simulink model "mijo"  (R2026b)
settings: Solver=VariableStepAuto  StopTime=15.0  MaxStep=1E-2
libraries: slpidlib x2
settings Model: LastModifiedBy=Emiliano
settings DataIOCC: DSMLogging=off  ReturnWorkspaceOutputs=off  SaveOutput=off  SignalLogging=off  TimeSaveName=t
settings DebuggingCC: AlgebraicLoopMsg=none  ArtificialAlgebraicLoopMsg=none  MaxConsecutiveZCsMsg=none

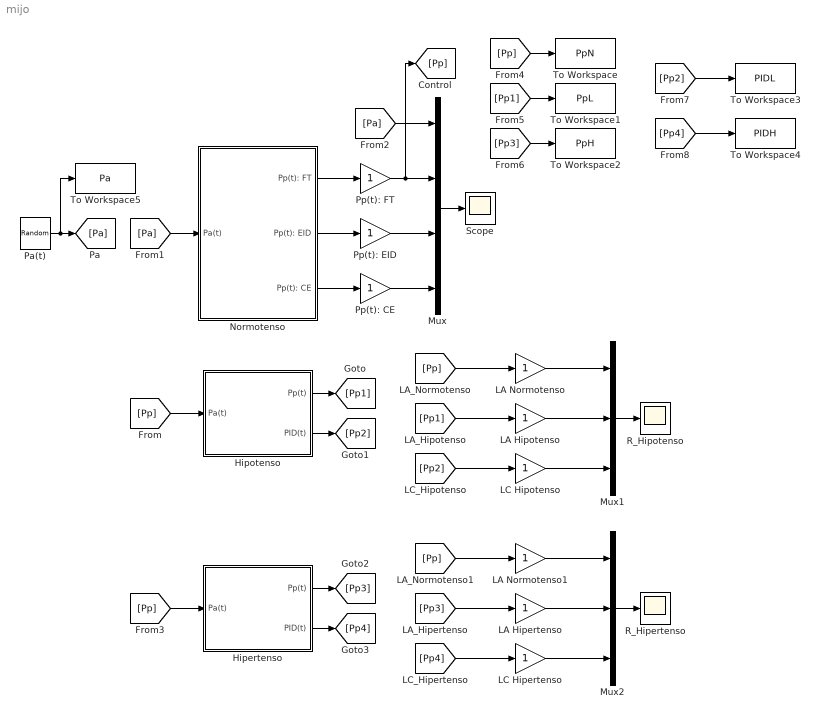
== system mijo ==
  Hipertenso : Subsystem
  Hipotenso : Subsystem
  LA Hipertenso : Gain
  LA Hipotenso : Gain
  LA Normotenso : Gain
  LA Normotenso1 : Gain
  LC Hipertenso : Gain
  LC Hipotenso : Gain
  Mux : Mux
  Mux1 : Mux  Inputs=3
  Mux2 : Mux  Inputs=3
  Normotenso : Subsystem
  Pa(t) : UniformRandomNumber  Minimum=-0.2  Seed=106  SampleTime=0.1
  Pp(t): CE : Gain
  Pp(t): EID : Gain
  Pp(t): FT : Gain
  R_Hipertenso : Scope
      settings: ActiveDisplayYMinimum=-0.45088607175795514  ActiveDisplayYMaximum=1.1087942936567985  DataLoggingVariableName=ScopeData2
  R_Hipotenso : Scope
      settings: ActiveDisplayYMinimum=0.091688488718673522  ActiveDisplayYMaximum=1.8821623827103118
  Scope : Scope
      settings: ActiveDisplayYMinimum=-0.51846261387700343  ActiveDisplayYMaximum=1.1468505763363619
  To Workspace : ToWorkspace  VariableName=PpN  SampleTime=-1
  To Workspace1 : ToWorkspace  VariableName=PpL  SampleTime=-1
  To Workspace2 : ToWorkspace  VariableName=PpH  SampleTime=-1
  To Workspace3 : ToWorkspace  VariableName=PIDL  SampleTime=-1
  To Workspace4 : ToWorkspace  VariableName=PIDH  SampleTime=-1
  To Workspace5 : ToWorkspace  VariableName=Pa  SampleTime=-1
  wires:
  Mux/1 -> Scope/1
  Normotenso/2(Pp(t): EID) -> Pp(t): EID/1
  Normotenso/3(Pp(t): CE) -> Pp(t): CE/1
  Normotenso/1(Pp(t): FT) -> Pp(t): FT/1
  Pp(t): FT/1 -> [Pp], Mux/2
  Pp(t): EID/1 -> Mux/3
  Pp(t): CE/1 -> Mux/4
  Pa(t)/1 -> To Workspace5/1, [Pa]
  [Pa] -> Normotenso/1(Pa(t))
  [Pa] -> Mux/1
  [Pp] -> Hipotenso/1(Pa(t))
  Hipotenso/1(Pp(t)) -> [Pp1]
  Hipotenso/2(PID(t)) -> [Pp2]
  [Pp] -> LA Normotenso/1
  [Pp1] -> LA Hipotenso/1
  [Pp2] -> LC Hipotenso/1
  Mux1/1 -> R_Hipotenso/1
  LA Normotenso/1 -> Mux1/1
  LA Hipotenso/1 -> Mux1/2
  LC Hipotenso/1 -> Mux1/3
  Hipertenso/2(PID(t)) -> [Pp4]
  Hipertenso/1(Pp(t)) -> [Pp3]
  [Pp] -> Hipertenso/1(Pa(t))
  LA Hipertenso/1 -> Mux2/2
  LA Normotenso1/1 -> Mux2/1
  Mux2/1 -> R_Hipertenso/1
  LC Hipertenso/1 -> Mux2/3
  [Pp4] -> LC Hipertenso/1
  [Pp3] -> LA Hipertenso/1
  [Pp] -> LA Normotenso1/1
  [Pp] -> To Workspace/1
  [Pp1] -> To Workspace1/1
  [Pp3] -> To Workspace2/1
  [Pp2] -> To Workspace3/1
  [Pp4] -> To Workspace4/1

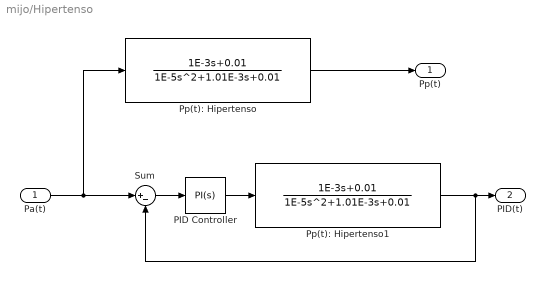
== system mijo/Hipertenso ==
  Pa(t) : Inport
  PID Controller : slpidlib/PID Controller  Controller=PI  Form=Parallel  TimeDomain=Continuous-time  UseExternalTs=off  SampleTime=-1  IntegratorMethod=Forward Euler  FilterMethod=Forward Euler  ControllerParametersSource=internal  P=205.8701  I=74187.5742  UseKiTs=off  D=0  UseExternalDerivativeSource=off  N=100  UseFilter=on  TunerSelectOption=Transfer Function Based (PID Tuner App)  InitialConditionSource=internal  InitialConditionForIntegrator=0  InitialConditionForFilter=0  DifferentiatorICPrevScaledInput=0  ExternalReset=none  TrackingMode=off  Kt=1  LimitOutput=off  SatLimitsSource=internal  UpperSaturationLimit=inf  LowerSaturationLimit=-inf  LinearizeAsGain=on  AntiWindupMode=none  Kb=1  LimitIntegrator=off  UpperIntegratorSaturationLimit=inf  LowerIntegratorSaturationLimit=-inf  POutMin=[]  POutMax=[]  IOutMin=[]  IOutMax=[]  DOutMin=[]  DOutMax=[]  NOutMin=[]  NOutMax=[]  SumOutMin=[]  SumOutMax=[]  SaturationOutMin=[]  SaturationOutMax=[]  PParamMin=[]  PParamMax=[]  IParamMin=[]  IParamMax=[]  DParamMin=[]  DParamMax=[]  NParamMin=[]  NParamMax=[]  KbParamMin=[]  KbParamMax=[]  KtParamMin=[]  KtParamMax=[]  KbOutMin=[]  KbOutMax=[]  KtOutMin=[]  KtOutMax=[]  IntegratorOutMin=[]  IntegratorOutMax=[]  FilterOutMin=[]  FilterOutMax=[]  SumI1OutMin=[]  SumI1OutMax=[]  SumI2OutMin=[]  SumI2OutMax=[]  SumI3OutMin=[]  SumI3OutMax=[]  SumI4OutMin=[]  SumI4OutMax=[]  SumDOutMin=[]  SumDOutMax=[]  DifferentiatorOutMin=[]  DifferentiatorOutMax=[]  FilterDiffOutCoefMin=[]  FilterDiffOutCoefMax=[]  ReciprocalOutMin=[]  ReciprocalOutMax=[]  SumDenOutMin=[]  SumDenOutMax=[]  SumNumOutMin=[]  SumNumOutMax=[]  DivideOutMin=[]  DivideOutMax=[]  UdiffTsProdOutMin=[]  UdiffTsProdOutMax=[]  NTsProdOutMin=[]  NTsProdOutMax=[]  UintegralTsProdOutMin=[]  UintegralTsProdOutMax=[]  UngainTsProdOutMin=[]  UngainTsProdOutMax=[]  ClampingZeroOutDataTypeStr=Inherit: Inherit via back propagation  ClampingZeroOutMin=[]  ClampingZeroOutMax=[]  FilterDenConstantOutDataTypeStr=Inherit: Inherit via back propagation  FilterDenConstantOutMin=[]  FilterDenConstantOutMax=[]  PCopyOutDataTypeStr=Inherit: Inherit via back propagation  PCopyOutMin=[]  PCopyOutMax=[]  NCopyOutDataTypeStr=Inherit: Inherit via back propagation  NCopyOutMin=[]  NCopyOutMax=[]  IntegratorContinuousStateAttributes=''  IntegratorStateMustResolveToSignalObject=off  IntegratorRTWStateStorageClass=Auto  FilterContinuousStateAttributes=''  FilterStateMustResolveToSignalObject=off  FilterRTWStateStorageClass=Auto  ParallelPVariant=InternalParameters  IdealPVariant=Disabled  IVariant=InternalParameters  DVariant=Disabled  IntegratorVariant=Continuous  SatVariant=Disabled  AWVariant=Passthrough  PCopyVariant=Disabled  TRVariant=Disabled  FdbkBlocksVariant=Forward  IdealPFdbkVariant=Disabled  SatFdbkVariant=Disabled  DerivativeFilterVariant=Disabled  NVariant=Disabled  NCopyVariant=Disabled_SignalSpec  FilterICVariant=Disabled  IntegratorICVariant=InternalICs  ExternalResetVariant=Disabled  TRSumVariant=Passthrough  SumFdbkVariant=Disabled  SumVariant=Sum_PI  TsampFilterVariant=InternalTs  TsampNgainVariant=Passthrough  TsampIntegralVariant=Disabled_SignalSpec  ExternalSaturationOutDataTypeStr=Inherit: Same as second input  DerivativeSourceVariant=Disabled  PreIntVariant=InternalPreInt
  Pp(t): Hipertenso : TransferFcn  Numerator=[1E-3,0.01]  Denominator=[1E-5,1.01E-3,0.01]
  Pp(t): Hipertenso1 : TransferFcn  Numerator=[1E-3,0.01]  Denominator=[1E-5,1.01E-3,0.01]
  Sum : Sum  Inputs=|+-
  Pp(t) : Outport
  PID(t) : Outport  Port=2
  wires:
  Pa(t)/1 -> Pp(t): Hipertenso/1, Sum/1
  PID Controller/1 -> Pp(t): Hipertenso1/1
  Sum/1 -> PID Controller/1
  Pp(t): Hipertenso1/1 -> Sum/2, PID(t)/1
  Pp(t): Hipertenso/1 -> Pp(t)/1

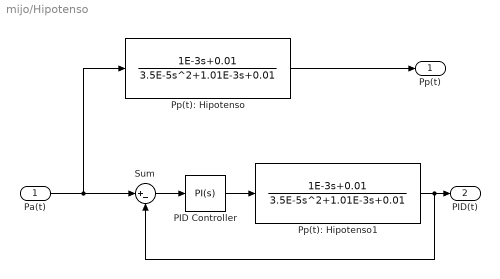
== system mijo/Hipotenso ==
  Pa(t) : Inport
  PID Controller : slpidlib/PID Controller  Controller=PI  Form=Parallel  TimeDomain=Continuous-time  UseExternalTs=off  SampleTime=-1  IntegratorMethod=Forward Euler  FilterMethod=Forward Euler  ControllerParametersSource=internal  P=174.4048  I=15212.346  UseKiTs=off  D=0  UseExternalDerivativeSource=off  N=100  UseFilter=on  TunerSelectOption=Transfer Function Based (PID Tuner App)  InitialConditionSource=internal  InitialConditionForIntegrator=0  InitialConditionForFilter=0  DifferentiatorICPrevScaledInput=0  ExternalReset=none  TrackingMode=off  Kt=1  LimitOutput=off  SatLimitsSource=internal  UpperSaturationLimit=inf  LowerSaturationLimit=-inf  LinearizeAsGain=on  AntiWindupMode=none  Kb=1  LimitIntegrator=off  UpperIntegratorSaturationLimit=inf  LowerIntegratorSaturationLimit=-inf  POutMin=[]  POutMax=[]  IOutMin=[]  IOutMax=[]  DOutMin=[]  DOutMax=[]  NOutMin=[]  NOutMax=[]  SumOutMin=[]  SumOutMax=[]  SaturationOutMin=[]  SaturationOutMax=[]  PParamMin=[]  PParamMax=[]  IParamMin=[]  IParamMax=[]  DParamMin=[]  DParamMax=[]  NParamMin=[]  NParamMax=[]  KbParamMin=[]  KbParamMax=[]  KtParamMin=[]  KtParamMax=[]  KbOutMin=[]  KbOutMax=[]  KtOutMin=[]  KtOutMax=[]  IntegratorOutMin=[]  IntegratorOutMax=[]  FilterOutMin=[]  FilterOutMax=[]  SumI1OutMin=[]  SumI1OutMax=[]  SumI2OutMin=[]  SumI2OutMax=[]  SumI3OutMin=[]  SumI3OutMax=[]  SumI4OutMin=[]  SumI4OutMax=[]  SumDOutMin=[]  SumDOutMax=[]  DifferentiatorOutMin=[]  DifferentiatorOutMax=[]  FilterDiffOutCoefMin=[]  FilterDiffOutCoefMax=[]  ReciprocalOutMin=[]  ReciprocalOutMax=[]  SumDenOutMin=[]  SumDenOutMax=[]  SumNumOutMin=[]  SumNumOutMax=[]  DivideOutMin=[]  DivideOutMax=[]  UdiffTsProdOutMin=[]  UdiffTsProdOutMax=[]  NTsProdOutMin=[]  NTsProdOutMax=[]  UintegralTsProdOutMin=[]  UintegralTsProdOutMax=[]  UngainTsProdOutMin=[]  UngainTsProdOutMax=[]  ClampingZeroOutDataTypeStr=Inherit: Inherit via back propagation  ClampingZeroOutMin=[]  ClampingZeroOutMax=[]  FilterDenConstantOutDataTypeStr=Inherit: Inherit via back propagation  FilterDenConstantOutMin=[]  FilterDenConstantOutMax=[]  PCopyOutDataTypeStr=Inherit: Inherit via back propagation  PCopyOutMin=[]  PCopyOutMax=[]  NCopyOutDataTypeStr=Inherit: Inherit via back propagation  NCopyOutMin=[]  NCopyOutMax=[]  IntegratorContinuousStateAttributes=''  IntegratorStateMustResolveToSignalObject=off  IntegratorRTWStateStorageClass=Auto  FilterContinuousStateAttributes=''  FilterStateMustResolveToSignalObject=off  FilterRTWStateStorageClass=Auto  ParallelPVariant=InternalParameters  IdealPVariant=Disabled  IVariant=InternalParameters  DVariant=Disabled  IntegratorVariant=Continuous  SatVariant=Disabled  AWVariant=Passthrough  PCopyVariant=Disabled  TRVariant=Disabled  FdbkBlocksVariant=Forward  IdealPFdbkVariant=Disabled  SatFdbkVariant=Disabled  DerivativeFilterVariant=Disabled  NVariant=Disabled  NCopyVariant=Disabled_SignalSpec  FilterICVariant=Disabled  IntegratorICVariant=InternalICs  ExternalResetVariant=Disabled  TRSumVariant=Passthrough  SumFdbkVariant=Disabled  SumVariant=Sum_PI  TsampFilterVariant=InternalTs  TsampNgainVariant=Passthrough  TsampIntegralVariant=Disabled_SignalSpec  ExternalSaturationOutDataTypeStr=Inherit: Same as second input  DerivativeSourceVariant=Disabled  PreIntVariant=InternalPreInt
  Pp(t): Hipotenso : TransferFcn  Numerator=[1E-3,0.01]  Denominator=[3.5E-5,1.01E-3,0.01]
  Pp(t): Hipotenso1 : TransferFcn  Numerator=[1E-3,0.01]  Denominator=[3.5E-5,1.01E-3,0.01]
  Sum : Sum  Inputs=|+-
  Pp(t) : Outport
  PID(t) : Outport  Port=2
  wires:
  Pa(t)/1 -> Sum/1, Pp(t): Hipotenso/1
  PID Controller/1 -> Pp(t): Hipotenso1/1
  Sum/1 -> PID Controller/1
  Pp(t): Hipotenso1/1 -> Sum/2, PID(t)/1
  Pp(t): Hipotenso/1 -> Pp(t)/1

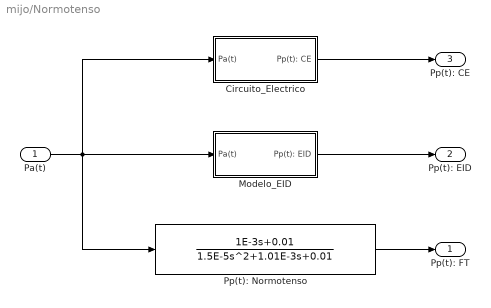
== system mijo/Normotenso ==
  Pa(t) : Inport
  Circuito_Electrico : Subsystem
  Modelo_EID : Subsystem
  Pp(t): Normotenso : TransferFcn  Numerator=[1E-3,0.01]  Denominator=[1.5E-5,1.01E-3,0.01]
  Pp(t): FT : Outport
  Pp(t): EID : Outport  Port=2
  Pp(t): CE : Outport  Port=3
  wires:
  Circuito_Electrico/1(Pp(t): CE) -> Pp(t): CE/1
  Modelo_EID/1(Pp(t): EID) -> Pp(t): EID/1
  Pa(t)/1 -> Pp(t): Normotenso/1, Modelo_EID/1(Pa(t)), Circuito_Electrico/1(Pa(t))
  Pp(t): Normotenso/1 -> Pp(t): FT/1

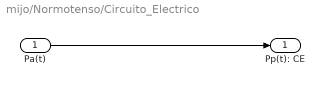
== system mijo/Normotenso/Circuito_Electrico ==
  Pa(t) : Inport
  Pp(t): CE : Outport
  wires:
  Pa(t)/1 -> Pp(t): CE/1

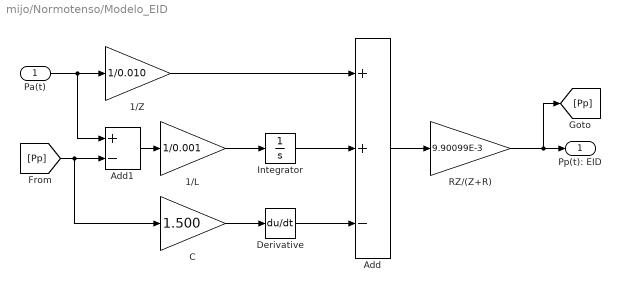
== system mijo/Normotenso/Modelo_EID ==
  Pa(t) : Inport
  1/L : Gain  Gain=1/0.001
  1/Z : Gain  Gain=1/0.010
  Add : Sum  Inputs=++-
  Add1 : Sum  Inputs=+-
  C : Gain  Gain=1.500
  Derivative : Derivative
  Integrator : Integrator
  RZ/(Z+R) : Gain  Gain=9.90099E-3
  Pp(t): EID : Outport
  wires:
  RZ/(Z+R)/1 -> [Pp], Pp(t): EID/1
  Add/1 -> RZ/(Z+R)/1
  Pa(t)/1 -> Add1/1, 1/Z/1
  1/Z/1 -> Add/1
  [Pp] -> C/1, Add1/2
  Add1/1 -> 1/L/1
  1/L/1 -> Integrator/1
  Integrator/1 -> Add/2
  C/1 -> Derivative/1
  Derivative/1 -> Add/3
